simulink model "pmpc_base"  (R2024b)
settings: Solver=ode1  StartTime=0.0  StopTime=3  FixedStep=0.001  RelTol=1e-3
InitFcn:
  | pmpc_base_setup('D:\OneDrive - mail.scut.edu.cn\Thesis\Code\Controller\Baseline\baseline_mpc')
values from neighbouring files (symbols this model uses):
  params = struct('M', M, 'vehicle', V, 'road', Road,                  'tireF', TireF, 'tireR', TireR)    [pmpc_base_init.m]    (also in run_baseline.m = evalin('base', 'params'))
  Reftraj = [(1:numel(X))', X, Y, unwrap(heading), curvature,             zeros(numel(X),1), station]    [pmpc_base_init.m]
  state0 = struct(      'u_prev',       zeros(2,1),      'plan',         zeros(2*M.Nc,1),      'path_index',   1,      'sw_prev',      0,      'brake_prev',   zeros(4,1),      'active_main',  false(8*M.Nc + 10*M.Np + 8,1),      'active_brake', false(8,1))    [pmpc_base_init.m]
undefined symbols (not defined in the file or in its folder): a_pl, b_pl, base_vtarget, dspblkCoreblockFVToolHelper, gcbh, Iref_init, Ki, Kp, Tc, Ts_avg
libraries: slpidlib x5, Solver_SF x1
settings Model: Creator=user  LastModifiedBy=user

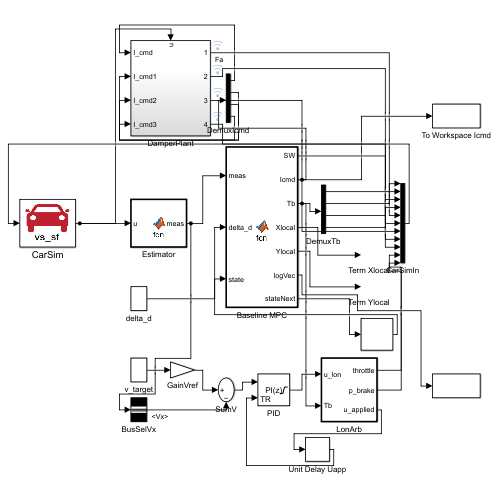
[thumbnail: Simulink's stored preview of the top-level diagram]
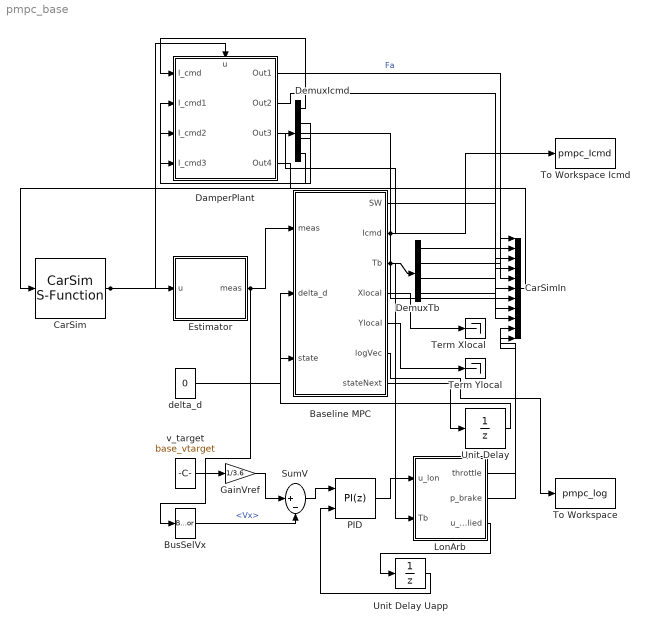
== system pmpc_base ==
  Baseline MPC : MATLAB Function  TreatAsAtomicUnit=on
  BusSelVx : BusSelector  OutputSignals=Vx
  CarSim : Solver_SF/CarSim S-Function  Priority=1  SIMFILE=D:\OneDrive - mail.scut.edu.cn\Thesis\Code\Jturn\simfile_dlc.sim
  CarSimIn : Mux  Inputs=11
  DamperPlant : Subsystem
      settings: PortSchema="{\"entries\":[{\"content\":{\"sides\":[{\"content\":{\"connectorIds\":[\"In1\",\"In2\",\"In3\",\"In4\"]},\"type\":\"ConnectorPlacement.EquallySpacedRectSide\",\"uuid\":\"6bdae15d-f673-492b-8508-25b25c52f85c\"},{\"content\":{\"connectorIds\":[\"Out1\",\"Out2\",\"Out3\",\"Out4\"],\"side\":\"RIGHT\"},\"type\":\"ConnectorPlacement.EquallySpacedRectSide\",\"uuid\":\"9d0d46be-4d90-4429-bc90-e3747ae06ca5\"},{\"content\":{\"connectorIds\":[\"In5\"],\"side\":\"TOP\"},\"type\":\"ConnectorPlacement.EquallySpacedRectSide\",\"uuid\":\"d2f3a784-c5ed-41f2-ae04-a2222bae6aeb\"}]},\"type\":\"ConnectorPlacement.EquallySpacedConnector\",\"uuid\":\"c35c18e7-51b3-4d33-8294-a9e611d66578\"}],\"packageUris\":[\"http://schema.mathworks.com/mf0/Connector/R2020b\"],\"version\":\"1.0\"}"
  DemuxIcmd : Demux
  DemuxTb : Demux
  Estimator : MATLAB Function  TreatAsAtomicUnit=on
  GainVref : Gain  Gain=1/3.6
  LonArb : MATLAB Function  TreatAsAtomicUnit=on
  PID : slpidlib/PID Controller  Controller=PI  Form=Parallel  TimeDomain=Discrete-time  UseExternalTs=off  SampleTime=0.01  IntegratorMethod=Forward Euler  FilterMethod=Forward Euler  ControllerParametersSource=internal  P=0.2  I=0.005  UseKiTs=off  D=0  UseExternalDerivativeSource=off  N=100  UseFilter=on  TunerSelectOption=Transfer Function Based (PID Tuner App)  InitialConditionSource=internal  InitialConditionForIntegrator=0  InitialConditionForFilter=0  DifferentiatorICPrevScaledInput=0  ExternalReset=none  TrackingMode=on  Kt=1  LimitOutput=on  SatLimitsSource=internal  UpperSaturationLimit=1  LowerSaturationLimit=-1  LinearizeAsGain=on  AntiWindupMode=back-calculation  Kb=1  LimitIntegrator=off  UpperIntegratorSaturationLimit=inf  LowerIntegratorSaturationLimit=-inf  POutMin=[]  POutMax=[]  IOutMin=[]  IOutMax=[]  DOutMin=[]  DOutMax=[]  NOutMin=[]  NOutMax=[]  SumOutMin=[]  SumOutMax=[]  SaturationOutMin=[]  SaturationOutMax=[]  PParamMin=[]  PParamMax=[]  IParamMin=[]  IParamMax=[]  DParamMin=[]  DParamMax=[]  NParamMin=[]  NParamMax=[]  KbParamMin=[]  KbParamMax=[]  KtParamMin=[]  KtParamMax=[]  KbOutMin=[]  KbOutMax=[]  KtOutMin=[]  KtOutMax=[]  IntegratorOutMin=[]  IntegratorOutMax=[]  FilterOutMin=[]  FilterOutMax=[]  SumI1OutMin=[]  SumI1OutMax=[]  SumI2OutMin=[]  SumI2OutMax=[]  SumI3OutMin=[]  SumI3OutMax=[]  SumI4OutMin=[]  SumI4OutMax=[]  SumDOutMin=[]  SumDOutMax=[]  DifferentiatorOutMin=[]  DifferentiatorOutMax=[]  FilterDiffOutCoefMin=[]  FilterDiffOutCoefMax=[]  ReciprocalOutMin=[]  ReciprocalOutMax=[]  SumDenOutMin=[]  SumDenOutMax=[]  SumNumOutMin=[]  SumNumOutMax=[]  DivideOutMin=[]  DivideOutMax=[]  UdiffTsProdOutMin=[]  UdiffTsProdOutMax=[]  NTsProdOutMin=[]  NTsProdOutMax=[]  UintegralTsProdOutMin=[]  UintegralTsProdOutMax=[]  UngainTsProdOutMin=[]  UngainTsProdOutMax=[]  ClampingZeroOutDataTypeStr=Inherit: Inherit via back propagation  ClampingZeroOutMin=[]  ClampingZeroOutMax=[]  FilterDenConstantOutDataTypeStr=Inherit: Inherit via back propagation  FilterDenConstantOutMin=[]  FilterDenConstantOutMax=[]  PCopyOutDataTypeStr=Inherit: Inherit via back propagation  PCopyOutMin=[]  PCopyOutMax=[]  NCopyOutDataTypeStr=Inherit: Inherit via back propagation  NCopyOutMin=[]  NCopyOutMax=[]  IntegratorContinuousStateAttributes=''  IntegratorStateMustResolveToSignalObject=off  IntegratorRTWStateStorageClass=Auto  FilterContinuousStateAttributes=''  FilterStateMustResolveToSignalObject=off  FilterRTWStateStorageClass=Auto  ParallelPVariant=InternalParameters  IdealPVariant=Disabled  IVariant=InternalParameters  DVariant=Disabled  IntegratorVariant=Discrete  SatVariant=Enabled  AWVariant=BackCalculation  PCopyVariant=Disabled  TRVariant=Enabled  FdbkBlocksVariant=Forward  IdealPFdbkVariant=Disabled  SatFdbkVariant=Disabled  DerivativeFilterVariant=Disabled  NVariant=Disabled  NCopyVariant=Disabled_SignalSpec  FilterICVariant=Disabled  IntegratorICVariant=InternalICs  ExternalResetVariant=Disabled  TRSumVariant=TrackingMode  SumFdbkVariant=Disabled  SumVariant=Sum_PI  TsampFilterVariant=InternalTs  TsampNgainVariant=Passthrough  TsampIntegralVariant=Disabled_SignalSpec  ExternalSaturationOutDataTypeStr=Inherit: Same as second input  DerivativeSourceVariant=Disabled  PreIntVariant=InternalPreInt
  SumV : Sum  Inputs=|+-
  Term Xlocal : Terminator
  Term Ylocal : Terminator
  To Workspace : ToWorkspace  VariableName=pmpc_log  SaveFormat=Timeseries  SampleTime=-1
  To Workspace Icmd : ToWorkspace  VariableName=pmpc_Icmd  SaveFormat=Structure With Time  SampleTime=-1
  Unit Delay : UnitDelay  InitialCondition=state0  SampleTime=0.01  HasFrameUpgradeWarning=on
  Unit Delay Uapp : UnitDelay  SampleTime=0.01  HasFrameUpgradeWarning=on
  delta_d : Constant  Value=0
  v_target : Constant  Value=base_vtarget
  wires:
  CarSim/1 -> Estimator/1(u), DamperPlant/5(u)
  Estimator/1(meas) -> Baseline MPC/1(meas), BusSelVx/1
  delta_d/1 -> Baseline MPC/2(delta_d)
  Unit Delay/1 -> Baseline MPC/3(state)
  Baseline MPC/4(Xlocal) -> Term Xlocal/1
  Baseline MPC/5(Ylocal) -> Term Ylocal/1
  Baseline MPC/6(logVec) -> To Workspace/1
  Baseline MPC/7(stateNext) -> Unit Delay/1
  Baseline MPC/2(Icmd) -> DemuxIcmd/1, To Workspace Icmd/1
  DemuxIcmd/1 -> DamperPlant/1(I_cmd)
  DamperPlant/1(Out1) -> CarSimIn/5  "Fa"
  DemuxIcmd/2 -> DamperPlant/2(I_cmd1)
  DamperPlant/2(Out2) -> CarSimIn/6
  DemuxIcmd/3 -> DamperPlant/3(I_cmd2)
  DamperPlant/3(Out3) -> CarSimIn/7
  DemuxIcmd/4 -> DamperPlant/4(I_cmd3)
  DamperPlant/4(Out4) -> CarSimIn/8
  Baseline MPC/3(Tb) -> DemuxTb/1, LonArb/2(Tb)
  DemuxTb/1 -> CarSimIn/1
  DemuxTb/2 -> CarSimIn/2
  DemuxTb/3 -> CarSimIn/3
  DemuxTb/4 -> CarSimIn/4
  Baseline MPC/1(SW) -> CarSimIn/9
  v_target/1 -> GainVref/1
  GainVref/1 -> SumV/1
  BusSelVx/1 -> SumV/2  "<Vx>"
  SumV/1 -> PID/1
  PID/1 -> LonArb/1(u_lon)
  LonArb/1(throttle) -> CarSimIn/10
  LonArb/2(p_brake) -> CarSimIn/11
  LonArb/3(u_applied) -> Unit Delay Uapp/1
  Unit Delay Uapp/1 -> PID/2
  CarSimIn/1 -> CarSim/1

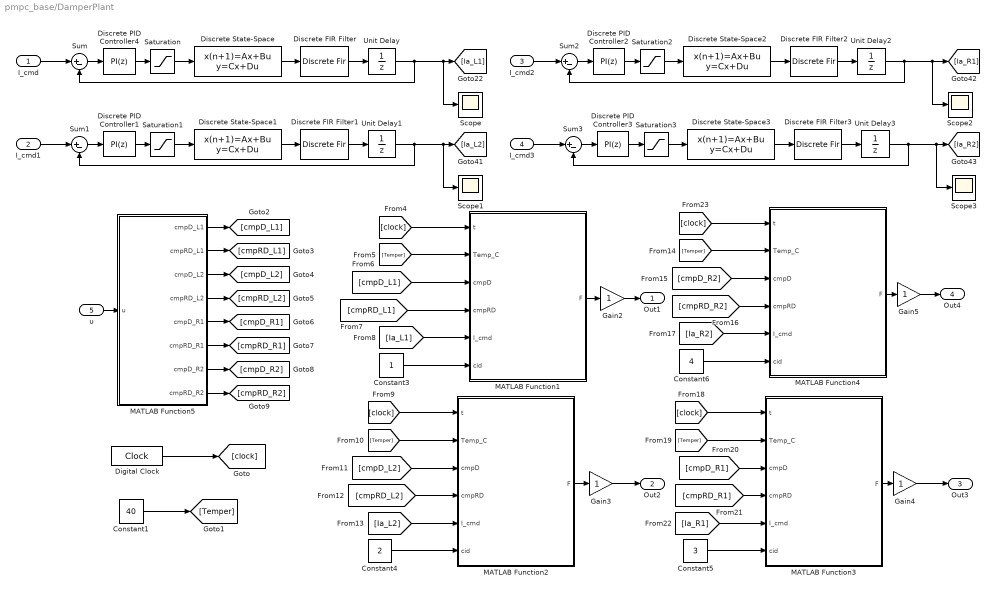
== system pmpc_base/DamperPlant ==
  I_cmd : Inport
  I_cmd1 : Inport  Port=2
  I_cmd2 : Inport  Port=3
  I_cmd3 : Inport  Port=4
  u : Inport  Port=5
  Constant1 : Constant  Value=40
  Constant3 : Constant
  Constant4 : Constant  Value=2
  Constant5 : Constant  Value=3
  Constant6 : Constant  Value=4
  Digital Clock : DigitalClock  SampleTime=0.001
  Discrete FIR Filter{,1..3} (4 alike) : DiscreteFir  LoadFcn=dspblkCoreblockFVToolHelper(gcbh,'load');  InitialStates=Iref_init
      settings: CopyFcn=dspblkCoreblockFVToolHelper(gcbh,'copy');  DeleteFcn=dspblkCoreblockFVToolHelper(gcbh,'close');  ModelCloseFcn=dspblkCoreblockFVToolHelper(gcbh,'close');  PreSaveFcn=dspblkCoreblockFVToolHelper(gcbh,'presave');  PostSaveFcn=dspblkCoreblockFVToolHelper(gcbh,'postsave');  CloseFcn=dspblkCoreblockFVToolHelper(gcbh,'close');
  Discrete PID Controller{1..4} (4 alike) : slpidlib/PID Controller  Controller=PI  Form=Parallel  TimeDomain=Discrete-time  UseExternalTs=off  SampleTime=Tc  IntegratorMethod=Forward Euler  FilterMethod=Forward Euler  ControllerParametersSource=internal  P=Kp  I=Ki  UseKiTs=off  D=0  UseExternalDerivativeSource=off  N=100  UseFilter=on  TunerSelectOption=Transfer Function Based (PID Tuner App)  InitialConditionSource=internal  InitialConditionForIntegrator=D_init  InitialConditionForFilter=0  DifferentiatorICPrevScaledInput=0  ExternalReset=none  TrackingMode=off  Kt=1  LimitOutput=on  SatLimitsSource=internal  UpperSaturationLimit=1  LowerSaturationLimit=0  LinearizeAsGain=off  AntiWindupMode=clamping  Kb=1  LimitIntegrator=off  UpperIntegratorSaturationLimit=duty_max − u_ff  LowerIntegratorSaturationLimit=duty_min − u_ff  POutMin=[]  POutMax=[]  IOutMin=[]  IOutMax=[]  DOutMin=[]  DOutMax=[]  NOutMin=[]  NOutMax=[]  SumOutMin=[]  SumOutMax=[]  SaturationOutMin=[]  SaturationOutMax=[]  PParamMin=[]  PParamMax=[]  IParamMin=[]  IParamMax=[]  DParamMin=[]  DParamMax=[]  NParamMin=[]  NParamMax=[]  KbParamMin=[]  KbParamMax=[]  KtParamMin=[]  KtParamMax=[]  KbOutMin=[]  KbOutMax=[]  KtOutMin=[]  KtOutMax=[]  IntegratorOutMin=[]  IntegratorOutMax=[]  FilterOutMin=[]  FilterOutMax=[]  SumI1OutMin=[]  SumI1OutMax=[]  SumI2OutMin=[]  SumI2OutMax=[]  SumI3OutMin=[]  SumI3OutMax=[]  SumI4OutMin=[]  SumI4OutMax=[]  SumDOutMin=[]  SumDOutMax=[]  DifferentiatorOutMin=[]  DifferentiatorOutMax=[]  FilterDiffOutCoefMin=[]  FilterDiffOutCoefMax=[]  ReciprocalOutMin=[]  ReciprocalOutMax=[]  SumDenOutMin=[]  SumDenOutMax=[]  SumNumOutMin=[]  SumNumOutMax=[]  DivideOutMin=[]  DivideOutMax=[]  UdiffTsProdOutMin=[]  UdiffTsProdOutMax=[]  NTsProdOutMin=[]  NTsProdOutMax=[]  UintegralTsProdOutMin=[]  UintegralTsProdOutMax=[]  UngainTsProdOutMin=[]  UngainTsProdOutMax=[]  ClampingZeroOutDataTypeStr=Inherit: Inherit via back propagation  ClampingZeroOutMin=[]  ClampingZeroOutMax=[]  FilterDenConstantOutDataTypeStr=Inherit: Inherit via back propagation  FilterDenConstantOutMin=[]  FilterDenConstantOutMax=[]  PCopyOutDataTypeStr=Inherit: Inherit via back propagation  PCopyOutMin=[]  PCopyOutMax=[]  NCopyOutDataTypeStr=Inherit: Inherit via back propagation  NCopyOutMin=[]  NCopyOutMax=[]  IntegratorContinuousStateAttributes=''  IntegratorStateMustResolveToSignalObject=off  IntegratorRTWStateStorageClass=Auto  FilterContinuousStateAttributes=''  FilterStateMustResolveToSignalObject=off  FilterRTWStateStorageClass=Auto  ParallelPVariant=InternalParameters  IdealPVariant=Disabled  IVariant=InternalParameters  DVariant=Disabled  IntegratorVariant=Discrete  SatVariant=Enabled  AWVariant=DiscClampingParallel  PCopyVariant=Disabled  TRVariant=Disabled  FdbkBlocksVariant=Forward  IdealPFdbkVariant=Disabled  SatFdbkVariant=Disabled  DerivativeFilterVariant=Disabled  NVariant=Disabled  NCopyVariant=Disabled_SignalSpec  FilterICVariant=Disabled  IntegratorICVariant=InternalICs  ExternalResetVariant=Disabled  TRSumVariant=Passthrough  SumFdbkVariant=Disabled  SumVariant=Sum_PI  TsampFilterVariant=InternalTs  TsampNgainVariant=Passthrough  TsampIntegralVariant=Disabled_SignalSpec  ExternalSaturationOutDataTypeStr=Inherit: Same as second input  DerivativeSourceVariant=Disabled  PreIntVariant=InternalPreInt
      settings: LibrarySourceBlock=simulink/Discrete/Discrete PID Controller
  Discrete State-Space{,1..3} (4 alike) : DiscreteStateSpace  A=a_pl  B=b_pl  D=0  InitialCondition=Iref_init  SampleTime=Ts_avg
  Gain{2..5} (4 alike) : Gain
  MATLAB Function1 : MATLAB Function  TreatAsAtomicUnit=on
  MATLAB Function2 : MATLAB Function  TreatAsAtomicUnit=on
  MATLAB Function3 : MATLAB Function  TreatAsAtomicUnit=on
  MATLAB Function4 : MATLAB Function  TreatAsAtomicUnit=on
  MATLAB Function5 : MATLAB Function  TreatAsAtomicUnit=on
  Saturation{,1..3} (4 alike) : Saturate  UpperLimit=1  LowerLimit=0
  Scope{,1..3} (4 alike) : Scope
  Sum{,1..3} (4 alike) : Sum  Inputs=|+-
  Unit Delay{,1..3} (4 alike) : UnitDelay  InitialCondition=Iref_init  SampleTime=1e-3  HasFrameUpgradeWarning=on
  Out1 : Outport
  Out2 : Outport  Port=2
  Out3 : Outport  Port=3
  Out4 : Outport  Port=4
  wires:
  I_cmd2/1 -> Sum2/1
  I_cmd1/1 -> Sum1/1
  Discrete PID Controller3/1 -> Saturation3/1
  I_cmd3/1 -> Sum3/1
  Sum3/1 -> Discrete PID Controller3/1
  Saturation3/1 -> Discrete State-Space3/1
  Discrete FIR Filter3/1 -> Unit Delay3/1
  Discrete State-Space3/1 -> Discrete FIR Filter3/1
  Unit Delay3/1 -> Sum3/2, Scope3/1, [Ia_R2]
  Discrete PID Controller2/1 -> Saturation2/1
  Sum2/1 -> Discrete PID Controller2/1
  Saturation2/1 -> Discrete State-Space2/1
  Discrete FIR Filter2/1 -> Unit Delay2/1
  Discrete State-Space2/1 -> Discrete FIR Filter2/1
  Unit Delay2/1 -> Sum2/2, Scope2/1, [Ia_R1]
  Discrete PID Controller1/1 -> Saturation1/1
  Sum1/1 -> Discrete PID Controller1/1
  Saturation1/1 -> Discrete State-Space1/1
  Discrete FIR Filter1/1 -> Unit Delay1/1
  Discrete State-Space1/1 -> Discrete FIR Filter1/1
  Unit Delay1/1 -> Sum1/2, Scope1/1, [Ia_L2]
  Saturation/1 -> Discrete State-Space/1
  Discrete State-Space/1 -> Discrete FIR Filter/1
  Discrete PID Controller4/1 -> Saturation/1
  Discrete FIR Filter/1 -> Unit Delay/1
  Unit Delay/1 -> Sum/2, [Ia_L1], Scope/1
  Sum/1 -> Discrete PID Controller4/1
  I_cmd/1 -> Sum/1
  MATLAB Function5/8(cmpRD_R2) -> [cmpRD_R2]
  MATLAB Function5/7(cmpD_R2) -> [cmpD_R2]
  MATLAB Function5/6(cmpRD_R1) -> [cmpRD_R1]
  MATLAB Function5/5(cmpD_R1) -> [cmpD_R1]
  MATLAB Function5/4(cmpRD_L2) -> [cmpRD_L2]
  MATLAB Function5/3(cmpD_L2) -> [cmpD_L2]
  MATLAB Function5/2(cmpRD_L1) -> [cmpRD_L1]
  MATLAB Function5/1(cmpD_L1) -> [cmpD_L1]
  u/1 -> MATLAB Function5/1(u)
  [cmpD_L2] -> MATLAB Function2/3(cmpD)
  [clock] -> MATLAB Function2/1(t)
  [Temper] -> MATLAB Function4/2(Temp_C)
  Constant3/1 -> MATLAB Function1/6(cid)
  [Temper] -> MATLAB Function2/2(Temp_C)
  Constant6/1 -> MATLAB Function4/6(cid)
  Gain2/1 -> Out1/1
  [cmpD_L1] -> MATLAB Function1/3(cmpD)
  MATLAB Function4/1(F) -> Gain5/1
  [clock] -> MATLAB Function1/1(t)
  Gain4/1 -> Out3/1
  [cmpRD_R2] -> MATLAB Function4/4(cmpRD)
  [cmpD_R1] -> MATLAB Function3/3(cmpD)
  [cmpRD_L2] -> MATLAB Function2/4(cmpRD)
  Constant1/1 -> [Temper]
  MATLAB Function3/1(F) -> Gain4/1
  [Temper] -> MATLAB Function3/2(Temp_C)
  Gain5/1 -> Out4/1
  [cmpRD_L1] -> MATLAB Function1/4(cmpRD)
  Gain3/1 -> Out2/1
  Digital Clock/1 -> [clock]
  [cmpD_R2] -> MATLAB Function4/3(cmpD)
  MATLAB Function2/1(F) -> Gain3/1
  Constant4/1 -> MATLAB Function2/6(cid)
  [Ia_L2] -> MATLAB Function2/5(I_cmd)
  [clock] -> MATLAB Function3/1(t)
  [Ia_L1] -> MATLAB Function1/5(I_cmd)
  [Ia_R1] -> MATLAB Function3/5(I_cmd)
  [cmpRD_R1] -> MATLAB Function3/4(cmpRD)
  MATLAB Function1/1(F) -> Gain2/1
  [Temper] -> MATLAB Function1/2(Temp_C)
  Constant5/1 -> MATLAB Function3/6(cid)
  [Ia_R2] -> MATLAB Function4/5(I_cmd)
  [clock] -> MATLAB Function4/1(t)

== matlab function pmpc_base/Baseline MPC ==
  settings: updateMethod=DISCRETE  sampleTime=0.01
  data: meas input Bus: PMPC_Base_MeasBus; SW output double; delta_d input; state input Bus: PMPC_Base_StateBus; Icmd output double; Tb output double; Xlocal output; Ylocal output; logVec output; stateNext output Bus: PMPC_Base_StateBus; Reftraj parameter; params parameter
function [SW,Icmd,Tb,Xlocal,Ylocal,logVec,stateNext] = ...
    fcn(meas,delta_d,state, Reftraj, params) %#codegen
[SW,Icmd,Tb,stateNext,Xlocal,Ylocal,logVec] = ...
    pmpc_base_step(meas,Reftraj,params,state,delta_d);
end

== matlab function pmpc_base/Estimator ==
  data: u input; meas output Bus: PMPC_Base_MeasBus
function meas = fcn(u) %#codegen
u = double(u(:));
meas = struct('X',u(40),'Y',u(41),'Vx',u(42)/3.6,'Vy',u(43)/3.6, ...
    'yaw',u(39)*pi/180,'r',u(34)*pi/180, ...
    'phi',u(38)*pi/180,'p',u(33)*pi/180, ...
    'delta_front',[u(46);u(47)]*pi/180,'steering_wheel',u(48)*pi/180, ...
    'Fx',u(9:12),'Fy',u(13:16),'Fz',u(17:20), ...
    'Fd',u(21:24),'Td',u(29:32),'vd',u(1:4)/1000);
end

== matlab function pmpc_base/LonArb ==
  settings: updateMethod=DISCRETE  sampleTime=0.01
  data: u_lon input; throttle output; Tb input; p_brake output; u_applied output
function [throttle,p_brake,u_applied] = fcn(u_lon,Tb) %#codegen
[throttle,p_brake,u_applied] = lon_arbitrate(u_lon,Tb);
end

== matlab function pmpc_base/DamperPlant/MATLAB Function1 ==
  data: t input; F output; Temp_C input; cmpD input; cmpRD input; I_cmd input; cid input
function F = fwd_mf(t, Temp_C, cmpD, cmpRD, I_cmd, cid)
%#codegen
F = fwd_mf_impl(t, Temp_C, cmpD, cmpRD, I_cmd, cid);

== matlab function pmpc_base/DamperPlant/MATLAB Function2 ==
  data: t input; F output; Temp_C input; cmpD input; cmpRD input; I_cmd input; cid input
function F = fwd_mf(t, Temp_C, cmpD, cmpRD, I_cmd, cid)
%#codegen
F = fwd_mf_impl(t, Temp_C, cmpD, cmpRD, I_cmd, cid);

== matlab function pmpc_base/DamperPlant/MATLAB Function3 ==
  data: t input; F output; Temp_C input; cmpD input; cmpRD input; I_cmd input; cid input
function F = fwd_mf(t, Temp_C, cmpD, cmpRD, I_cmd, cid)
%#codegen
F = fwd_mf_impl(t, Temp_C, cmpD, cmpRD, I_cmd, cid);

== matlab function pmpc_base/DamperPlant/MATLAB Function4 ==
  data: t input; F output; Temp_C input; cmpD input; cmpRD input; I_cmd input; cid input
function F = fwd_mf(t, Temp_C, cmpD, cmpRD, I_cmd, cid)
%#codegen
F = fwd_mf_impl(t, Temp_C, cmpD, cmpRD, I_cmd, cid);

== matlab function pmpc_base/DamperPlant/MATLAB Function5 ==
  data: u input; cmpD_L1 output; cmpRD_L1 output; cmpD_L2 output; cmpRD_L2 output; cmpD_R1 output; cmpRD_R1 output; cmpD_R2 output; cmpRD_R2 output
function [cmpD_L1,cmpRD_L1,cmpD_L2,cmpRD_L2, ...
          cmpD_R1,cmpRD_R1,cmpD_R2,cmpRD_R2] = fcn(u)
%#codegen
% u：当前 CarSim 54 路输出
% 位移 mm，速度 mm/s，保持原单位

cmpD_L1  = u(51);
cmpRD_L1 = u(1);

cmpD_L2  = u(52);
cmpRD_L2 = u(2);

cmpD_R1  = u(53);
cmpRD_R1 = u(3);

cmpD_R2  = u(54);
cmpRD_R2 = u(4);
end
